simulink model "Sm_Ideal"  (R2025b)
settings: Solver=FixedStepDiscrete  StartTime=0.0  StopTime=0.1  FixedStep=Par_Sw_cdTs  RelTol=1e-3
undefined symbols (not defined in the file or in its folder): Par_Mtr_cfFlux, Par_Mtr_cfLd, Par_Mtr_cfLq, Par_Mtr_cfRs, Par_Mtr_cuNp, Par_Sw_cdTs
libraries: Lib_PMSMCtrl x3, eeTransforms x2
settings Model: DataDictionary=Sm_Ideal.sldd  SimulationMode=accelerator  Creator=62555  LastModifiedBy=62555
settings OptimizationCC: DefaultParameterBehavior=Inlined  UseDivisionForNetSlopeComputation=on  EnhancedBackFolding=on  PassReuseOutputArgsAs=Individual arguments  ZeroExternalMemoryAtStartup=off  ZeroInternalMemoryAtStartup=off  OptimizeBlockOrder=speed  DifferentSizesBufferReuse=on  OptimizationCustomize=off  EfficientTunableParamExpr=on
settings DebuggingCC: ParameterTunabilityLossMsg=error
settings SFSimCC: MATLABDynamicMemAlloc=off
settings RTWCC: SystemTargetFile=ert.tlc  GenCodeOnly=on  TemplateMakefile=ert_default_tmf  Toolchain=MinGW64 | gmake (64-bit Windows)  Description=Embedded Coder
settings CodeAppCC: ForceParamTrailComments=on  IgnoreCustomStorageClasses=off  OperatorAnnotations=on  SimulinkDataObjDesc=on  SFDataObjDesc=on  InsertBlockDesc=on
settings ERTTargetCC: ERTCustomFileTemplate=example_file_process.tlc  TargetLangStandard=C99 (ISO)  GenerateSampleERTMain=on

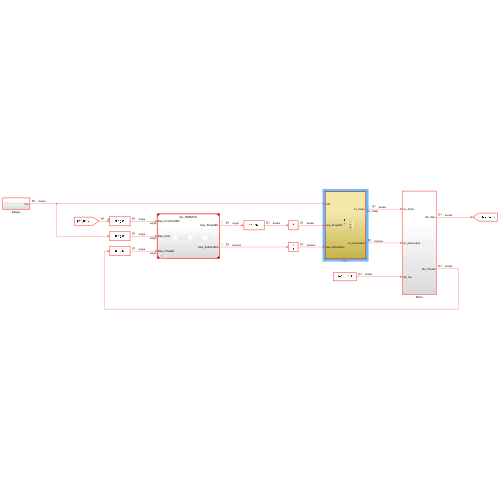
[thumbnail: Simulink's stored preview of the top-level diagram]
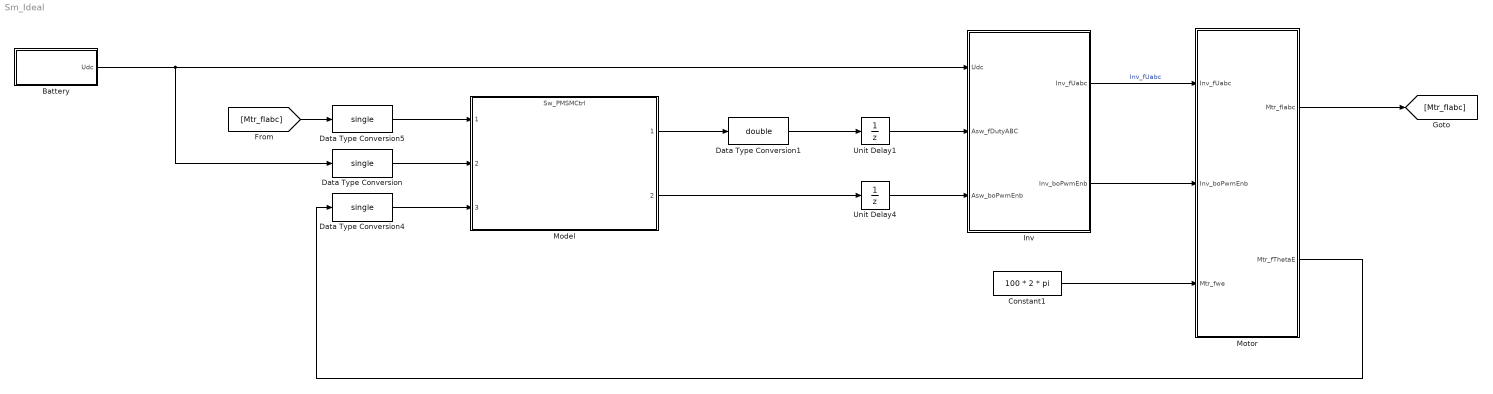
== system Sm_Ideal ==
  Battery : Subsystem
  Constant1 : Constant  Value=100 * 2 * pi  OutDataTypeStr=double  SampleTime=-1
  Data Type Conversion : DataTypeConversion  OutDataTypeStr=single  SaturateOnIntegerOverflow=off  RndMeth=Floor
  Data Type Conversion1 : DataTypeConversion  OutDataTypeStr=double  SaturateOnIntegerOverflow=off  RndMeth=Floor
  Data Type Conversion4 : DataTypeConversion  OutDataTypeStr=single  SaturateOnIntegerOverflow=off  RndMeth=Floor
  Data Type Conversion5 : DataTypeConversion  OutDataTypeStr=single  SaturateOnIntegerOverflow=off  RndMeth=Floor
  Inv : Subsystem
  Model : ModelReference  ModelNameDialog=Sw_PMSMCtrl.slx  ModelReferenceVersion=6.14
  Motor : Subsystem
  Unit Delay1 : UnitDelay  SampleTime=-1  HasFrameUpgradeWarning=on
  Unit Delay4 : UnitDelay  SampleTime=-1  HasFrameUpgradeWarning=on
  wires:
  Model/2 -> Unit Delay4/1
  Model/1 -> Data Type Conversion1/1
  Data Type Conversion/1 -> Model/2
  Data Type Conversion1/1 -> Unit Delay1/1
  Data Type Conversion4/1 -> Model/3
  Inv/2(Inv_boPwmEnb) -> Motor/2(Inv_boPwmEnb)
  Inv/1(Inv_fUabc) -> Motor/1(Inv_fUabc)  "Inv_fUabc"
  [Mtr_fIabc] -> Data Type Conversion5/1
  Data Type Conversion5/1 -> Model/1
  Motor/1(Mtr_fIabc) -> [Mtr_fIabc]
  Unit Delay1/1 -> Inv/2(Asw_fDutyABC)
  Unit Delay4/1 -> Inv/3(Asw_boPwmEnb)
  Battery/1(Udc) -> Inv/1(Udc), Data Type Conversion/1
  Constant1/1 -> Motor/3(Mtr_fwe)
  Motor/2(Mtr_fThetaE) -> Data Type Conversion4/1

== system Sm_Ideal/Battery ==
  Constant : Constant  Value=48  OutDataTypeStr=double  SampleTime=-1
  Udc : Outport
  wires:
  Constant/1 -> Udc/1

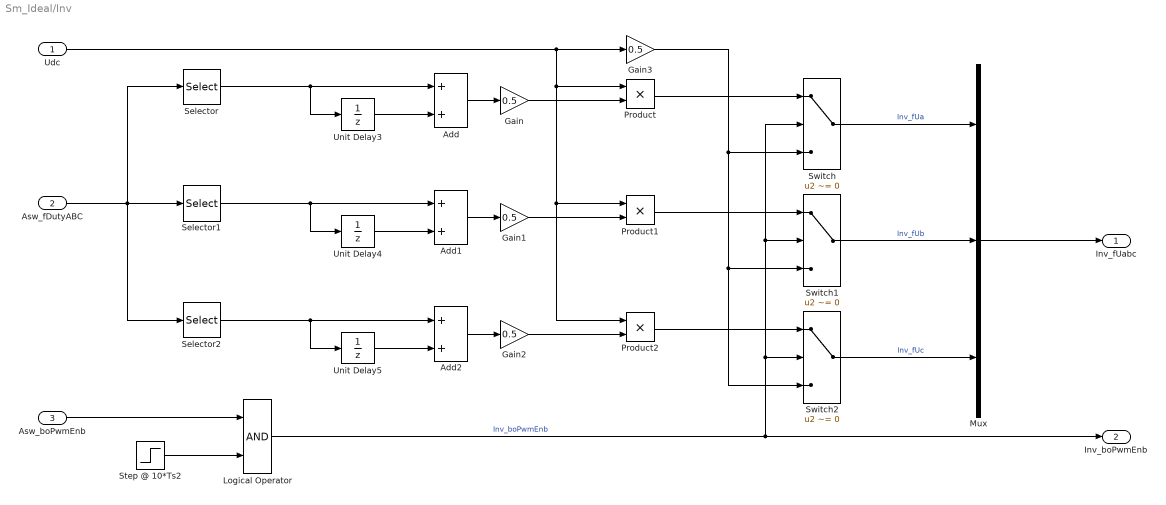
== system Sm_Ideal/Inv ==
  Udc : Inport
  Asw_fDutyABC : Inport  Port=2
  Asw_boPwmEnb : Inport  Port=3
  Add : Sum
  Add1 : Sum
  Add2 : Sum
  Gain{,1..3} (4 alike) : Gain  Gain=0.5
  Logical Operator : Logic  AllPortsSameDT=off  OutDataTypeStr=boolean
  Mux : Mux  Inputs=3
  Product : Product
  Product1 : Product
  Product2 : Product
  Selector : Selector  InputPortWidth=3  IndexOptions=Index vector (dialog)  Indices=[1]  OutputSizes=1
  Selector1 : Selector  InputPortWidth=3  IndexOptions=Index vector (dialog)  Indices=[2]  OutputSizes=1
  Selector2 : Selector  InputPortWidth=3  IndexOptions=Index vector (dialog)  Indices=[3]  OutputSizes=1
  Step @ 10*Ts2 : Step  Time=0.00050  SampleTime=Par_Sw_cdTs
  Switch : Switch  Criteria=u2 ~= 0  SaturateOnIntegerOverflow=off  InputSameDT=off
  Switch1 : Switch  Criteria=u2 ~= 0  SaturateOnIntegerOverflow=off  InputSameDT=off
  Switch2 : Switch  Criteria=u2 ~= 0  SaturateOnIntegerOverflow=off  InputSameDT=off
  Unit Delay3 : UnitDelay  SampleTime=-1  HasFrameUpgradeWarning=on
  Unit Delay4 : UnitDelay  SampleTime=-1  HasFrameUpgradeWarning=on
  Unit Delay5 : UnitDelay  SampleTime=-1  HasFrameUpgradeWarning=on
  Inv_fUabc : Outport
  Inv_boPwmEnb : Outport  Port=2
  wires:
  Udc/1 -> Gain3/1, Product2/1, Product1/1, Product/1
  Add/1 -> Gain/1
  Gain/1 -> Product/2
  Unit Delay3/1 -> Add/2
  Add1/1 -> Gain1/1
  Unit Delay4/1 -> Add1/2
  Add2/1 -> Gain2/1
  Unit Delay5/1 -> Add2/2
  Asw_fDutyABC/1 -> Selector/1, Selector2/1, Selector1/1
  Gain1/1 -> Product1/2
  Gain2/1 -> Product2/2
  Product/1 -> Switch/1
  Product1/1 -> Switch1/1
  Product2/1 -> Switch2/1
  Asw_boPwmEnb/1 -> Logical Operator/1
  Step @ 10*Ts2/1 -> Logical Operator/2
  Logical Operator/1 -> Switch1/2, Switch/2, Switch2/2, Inv_boPwmEnb/1  "Inv_boPwmEnb"
  Gain3/1 -> Switch2/3, Switch1/3, Switch/3
  Switch/1 -> Mux/1  "Inv_fUa"
  Switch2/1 -> Mux/3  "Inv_fUc"
  Switch1/1 -> Mux/2  "Inv_fUb"
  Mux/1 -> Inv_fUabc/1
  Selector/1 -> Unit Delay3/1, Add/1
  Selector1/1 -> Unit Delay4/1, Add1/1
  Selector2/1 -> Unit Delay5/1, Add2/1

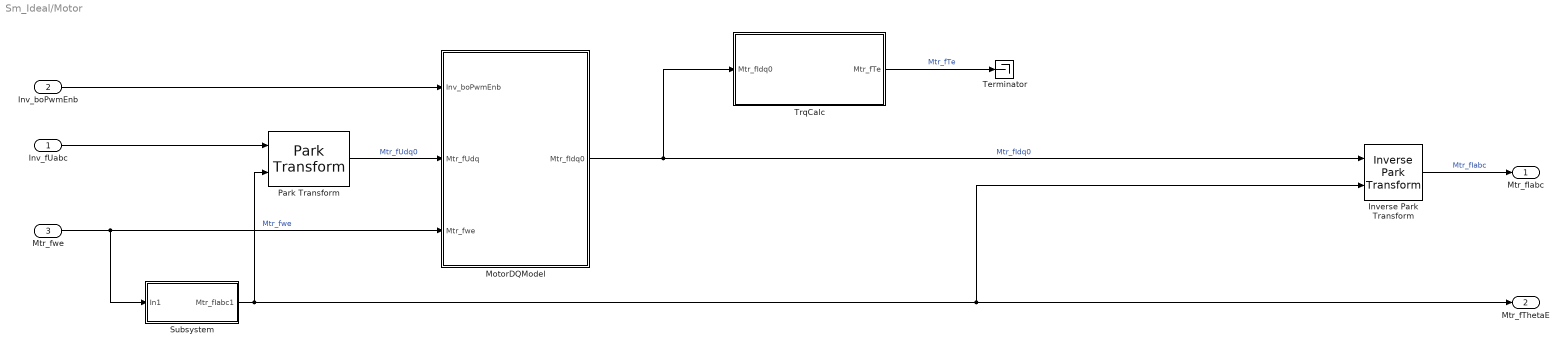
== system Sm_Ideal/Motor ==
  Inv_fUabc : Inport
  Inv_boPwmEnb : Inport  Port=2
  Mtr_fwe : Inport  Port=3
  Inverse Park Transform : eeTransforms/Inverse Park Transform  AxisAlignment=D-axis  PowerInvariant=off
      settings: LibrarySourceBlock=|
      | ee_sl_lib/Mathematical
      | Transforms/Inverse
      | Park Transform
  MotorDQModel : Subsystem  mask{Ld=Par_Mtr_cfLd, Lq=Par_Mtr_cfLq, Rs=Par_Mtr_cfRs, Psif=Par_Mtr_cfFlux}
      mask prompts: Ld "Ld (H)"; Lq "Lq (H)"; Rs "Rs (Ω)"; Psif "Psif (Wb)"
      mask Display:
      | disp('Motor Elec Model\n dq-Axis');
      | port_label('input',1, 'PwmEnb','interpreter', 'tex');
      | port_label('input',2, 'Udq0','interpreter', 'tex');
      | port_label('input',3, '\omega_e','interpreter', 'tex');
      | port_label('output',1, 'Idq0','interpreter', 'tex');
  Park Transform : eeTransforms/Park Transform  AxisAlignment=D-axis  PowerInvariant=off
      settings: LibrarySourceBlock=|
      | ee_sl_lib/Mathematical
      | Transforms/Park Transform
  Subsystem : Subsystem
  Terminator : Terminator
  TrqCalc : Subsystem
  Mtr_fIabc : Outport
  Mtr_fThetaE : Outport  Port=2
  wires:
  Mtr_fwe/1 -> Subsystem/1(In1), MotorDQModel/3(Mtr_fwe)  "Mtr_fwe"
  MotorDQModel/1(Mtr_fIdq0) -> TrqCalc/1(Mtr_fIdq0), Inverse Park Transform/1  "Mtr_fIdq0"
  Inv_boPwmEnb/1 -> MotorDQModel/1(Inv_boPwmEnb)
  Inv_fUabc/1 -> Park Transform/1
  Park Transform/1 -> MotorDQModel/2(Mtr_fUdq)  "Mtr_fUdq0"
  Inverse Park Transform/1 -> Mtr_fIabc/1  "Mtr_fIabc"
  TrqCalc/1(Mtr_fTe) -> Terminator/1  "Mtr_fTe"
  Subsystem/1(Mtr_fIabc1) -> Park Transform/2, Inverse Park Transform/2, Mtr_fThetaE/1

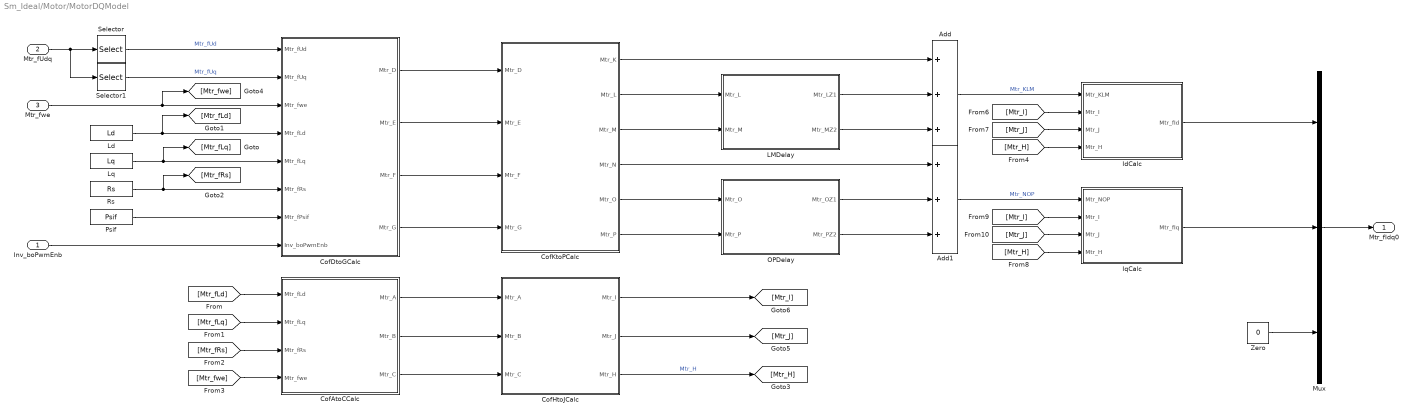
== system Sm_Ideal/Motor/MotorDQModel ==
  Inv_boPwmEnb : Inport
  Mtr_fUdq : Inport  Port=2
  Mtr_fwe : Inport  Port=3
  Add : Sum  Inputs=+++
  Add1 : Sum  Inputs=+++
  CofAtoCCalc : Subsystem
  CofDtoGCalc : Subsystem
  CofHtoJCalc : Subsystem
  CofKtoPCalc : Subsystem
  IdCalc : Subsystem
  IqCalc : Subsystem
  LMDelay : Subsystem
  Ld : Constant  Value=Ld  OutDataTypeStr=double  SampleTime=-1
  Lq : Constant  Value=Lq  OutDataTypeStr=double  SampleTime=-1
  Mux : Mux  Inputs=3
  OPDelay : Subsystem
  Psif : Constant  Value=Psif  OutDataTypeStr=double  SampleTime=-1
  Rs : Constant  Value=Rs  OutDataTypeStr=double  SampleTime=-1
  Selector : Selector  InputPortWidth=3  IndexOptions=Index vector (dialog)  Indices=[1]  OutputSizes=1
  Selector1 : Selector  InputPortWidth=3  IndexOptions=Index vector (dialog)  Indices=[2]  OutputSizes=1
  Zero : Constant  Value=0  OutDataTypeStr=Inherit: Inherit via back propagation
  Mtr_fIdq0 : Outport
  wires:
  [Mtr_fLd] -> CofAtoCCalc/1(Mtr_fLd)
  [Mtr_fLq] -> CofAtoCCalc/2(Mtr_fLq)
  [Mtr_fRs] -> CofAtoCCalc/3(Mtr_fRs)
  [Mtr_fwe] -> CofAtoCCalc/4(Mtr_fwe)
  Mtr_fwe/1 -> [Mtr_fwe], CofDtoGCalc/3(Mtr_fwe)
  Ld/1 -> CofDtoGCalc/4(Mtr_fLd), [Mtr_fLd]
  Lq/1 -> CofDtoGCalc/5(Mtr_fLq), [Mtr_fLq]
  Rs/1 -> [Mtr_fRs], CofDtoGCalc/6(Mtr_fRs)
  Psif/1 -> CofDtoGCalc/7(Mtr_fPsif)
  CofAtoCCalc/2(Mtr_B) -> CofHtoJCalc/2(Mtr_B)
  CofAtoCCalc/1(Mtr_A) -> CofHtoJCalc/1(Mtr_A)
  CofAtoCCalc/3(Mtr_C) -> CofHtoJCalc/3(Mtr_C)
  CofDtoGCalc/3(Mtr_F) -> CofKtoPCalc/3(Mtr_F)
  CofDtoGCalc/4(Mtr_G) -> CofKtoPCalc/4(Mtr_G)
  CofDtoGCalc/2(Mtr_E) -> CofKtoPCalc/2(Mtr_E)
  CofDtoGCalc/1(Mtr_D) -> CofKtoPCalc/1(Mtr_D)
  CofHtoJCalc/1(Mtr_I) -> [Mtr_I]
  CofHtoJCalc/2(Mtr_J) -> [Mtr_J]
  CofKtoPCalc/5(Mtr_O) -> OPDelay/1(Mtr_O)
  CofKtoPCalc/6(Mtr_P) -> OPDelay/2(Mtr_P)
  CofKtoPCalc/2(Mtr_L) -> LMDelay/1(Mtr_L)
  CofKtoPCalc/3(Mtr_M) -> LMDelay/2(Mtr_M)
  CofHtoJCalc/3(Mtr_H) -> [Mtr_H]  "Mtr_H"
  CofKtoPCalc/1(Mtr_K) -> Add/1
  CofKtoPCalc/4(Mtr_N) -> Add1/1
  LMDelay/1(Mtr_LZ1) -> Add/2
  LMDelay/2(Mtr_MZ2) -> Add/3
  OPDelay/1(Mtr_OZ1) -> Add1/2
  OPDelay/2(Mtr_PZ2) -> Add1/3
  Add/1 -> IdCalc/1(Mtr_KLM)  "Mtr_KLM"
  IdCalc/1(Mtr_fId) -> Mux/1
  [Mtr_H] -> IdCalc/4(Mtr_H)
  [Mtr_I] -> IdCalc/2(Mtr_I)
  [Mtr_J] -> IdCalc/3(Mtr_J)
  [Mtr_I] -> IqCalc/2(Mtr_I)
  [Mtr_J] -> IqCalc/3(Mtr_J)
  [Mtr_H] -> IqCalc/4(Mtr_H)
  Add1/1 -> IqCalc/1(Mtr_NOP)  "Mtr_NOP"
  IqCalc/1(Mtr_fIq) -> Mux/2
  Inv_boPwmEnb/1 -> CofDtoGCalc/8(Inv_boPwmEnb)
  Selector/1 -> CofDtoGCalc/1(Mtr_fUd)  "Mtr_fUd"
  Mtr_fUdq/1 -> Selector/1, Selector1/1
  Selector1/1 -> CofDtoGCalc/2(Mtr_fUq)  "Mtr_fUq"
  Mux/1 -> Mtr_fIdq0/1
  Zero/1 -> Mux/3

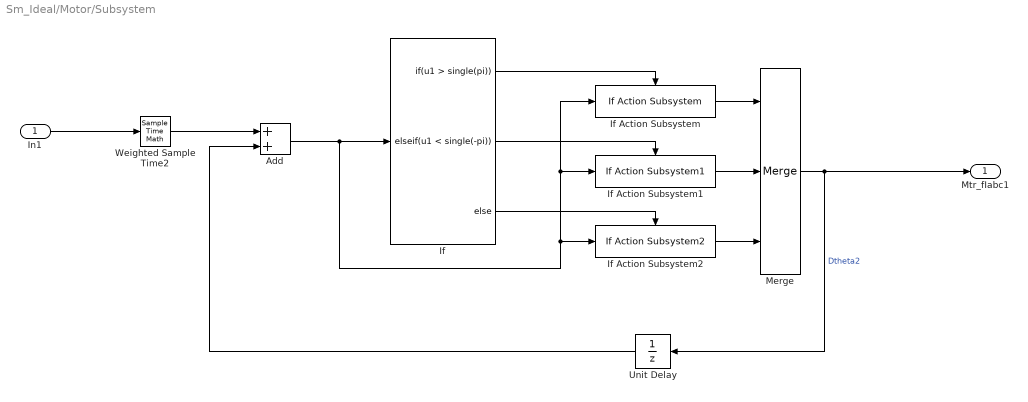
== system Sm_Ideal/Motor/Subsystem ==
  In1 : Inport
  Add : Sum
  If : If  IfExpression=u1 > single(pi)  ElseIfExpressions=u1 < single(-pi)
  If Action Subsystem : Lib_PMSMCtrl/PostoSpd/If Action Subsystem  SystemSampleTime=-1  VariantActivationTime=update diagram  EmptyChoice=off  PassThrough=off  PassThroughVariantControl=(default)  EmptyChoiceVariantControl=(default)  AllowFlexibleInterface=on  Latency=0  AutoFrameSizeCalculation=off
      settings: SourceProductName=Lib_PMSMCtrl
  If Action Subsystem1 : Lib_PMSMCtrl/PostoSpd/If Action Subsystem1  SystemSampleTime=-1  VariantActivationTime=update diagram  EmptyChoice=off  PassThrough=off  PassThroughVariantControl=(default)  EmptyChoiceVariantControl=(default)  AllowFlexibleInterface=on  Latency=0  AutoFrameSizeCalculation=off
      settings: SourceProductName=Lib_PMSMCtrl
  If Action Subsystem2 : Lib_PMSMCtrl/PostoSpd/If Action Subsystem2  SystemSampleTime=-1  VariantActivationTime=update diagram  EmptyChoice=off  PassThrough=off  PassThroughVariantControl=(default)  EmptyChoiceVariantControl=(default)  AllowFlexibleInterface=on  Latency=0  AutoFrameSizeCalculation=off
      settings: SourceProductName=Lib_PMSMCtrl
  Merge : Merge  Inputs=3
  Unit Delay : UnitDelay  SampleTime=-1  HasFrameUpgradeWarning=on
  Weighted Sample Time2 : SampleTimeMath  TsampMathOp=*
  Mtr_fIabc1 : Outport
  wires:
  If/3 -> If Action Subsystem2/Action
  If Action Subsystem/1 -> Merge/1
  If/2 -> If Action Subsystem1/Action
  Merge/1 -> Mtr_fIabc1/1, Unit Delay/1  "Dtheta2"
  If Action Subsystem2/1 -> Merge/3
  Weighted Sample Time2/1 -> Add/1
  Add/1 -> If Action Subsystem/1, If Action Subsystem1/1, If Action Subsystem2/1, If/1
  If/1 -> If Action Subsystem/Action
  If Action Subsystem1/1 -> Merge/2
  Unit Delay/1 -> Add/2
  In1/1 -> Weighted Sample Time2/1

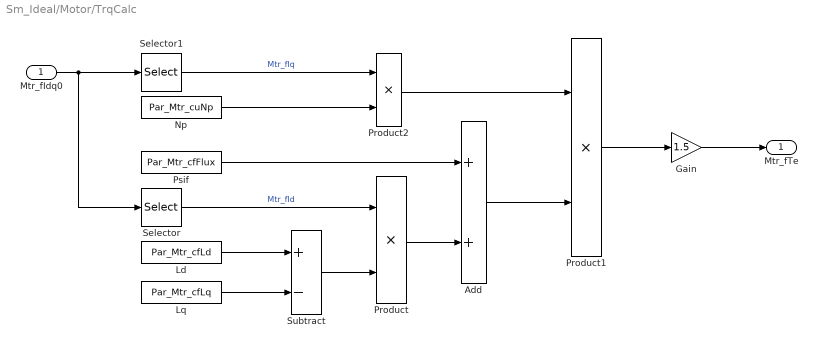
== system Sm_Ideal/Motor/TrqCalc ==
  Mtr_fIdq0 : Inport
  Add : Sum
  Gain : Gain  Gain=1.5
  Ld : Constant  Value=Par_Mtr_cfLd  OutDataTypeStr=double  SampleTime=-1
  Lq : Constant  Value=Par_Mtr_cfLq  OutDataTypeStr=double  SampleTime=-1
  Np : Constant  Value=Par_Mtr_cuNp  OutDataTypeStr=double  SampleTime=-1
  Product : Product
  Product1 : Product
  Product2 : Product
  Psif : Constant  Value=Par_Mtr_cfFlux  OutDataTypeStr=double  SampleTime=-1
  Selector : Selector  InputPortWidth=3  IndexOptions=Index vector (dialog)  Indices=[1]  OutputSizes=1
  Selector1 : Selector  InputPortWidth=3  IndexOptions=Index vector (dialog)  Indices=[2]  OutputSizes=1
  Subtract : Sum  Inputs=+-
  Mtr_fTe : Outport
  wires:
  Selector/1 -> Product/1  "Mtr_fId"
  Selector1/1 -> Product2/1  "Mtr_fIq"
  Mtr_fIdq0/1 -> Selector/1, Selector1/1
  Ld/1 -> Subtract/1
  Lq/1 -> Subtract/2
  Subtract/1 -> Product/2
  Product/1 -> Add/2
  Psif/1 -> Add/1
  Add/1 -> Product1/2
  Product1/1 -> Gain/1
  Gain/1 -> Mtr_fTe/1
  Product2/1 -> Product1/1
  Np/1 -> Product2/2

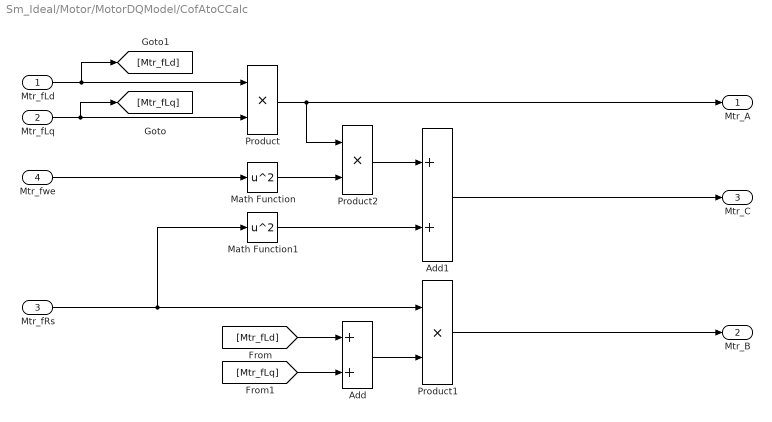
== system Sm_Ideal/Motor/MotorDQModel/CofAtoCCalc ==
  Mtr_fLd : Inport
  Mtr_fLq : Inport  Port=2
  Mtr_fRs : Inport  Port=3
  Mtr_fwe : Inport  Port=4
  Add : Sum
  Add1 : Sum
  Math Function : Math  Operator=square
  Math Function1 : Math  Operator=square
  Product : Product
  Product1 : Product
  Product2 : Product
  Mtr_A : Outport
  Mtr_B : Outport  Port=2
  Mtr_C : Outport  Port=3
  wires:
  Mtr_fLq/1 -> [Mtr_fLq], Product/2
  Mtr_fRs/1 -> Product1/1, Math Function1/1
  Product1/1 -> Mtr_B/1
  Mtr_fLd/1 -> [Mtr_fLd], Product/1
  Add1/1 -> Mtr_C/1
  Add/1 -> Product1/2
  [Mtr_fLd] -> Add/1
  [Mtr_fLq] -> Add/2
  Product2/1 -> Add1/1
  Mtr_fwe/1 -> Math Function/1
  Math Function/1 -> Product2/2
  Math Function1/1 -> Add1/2
  Product/1 -> Mtr_A/1, Product2/1

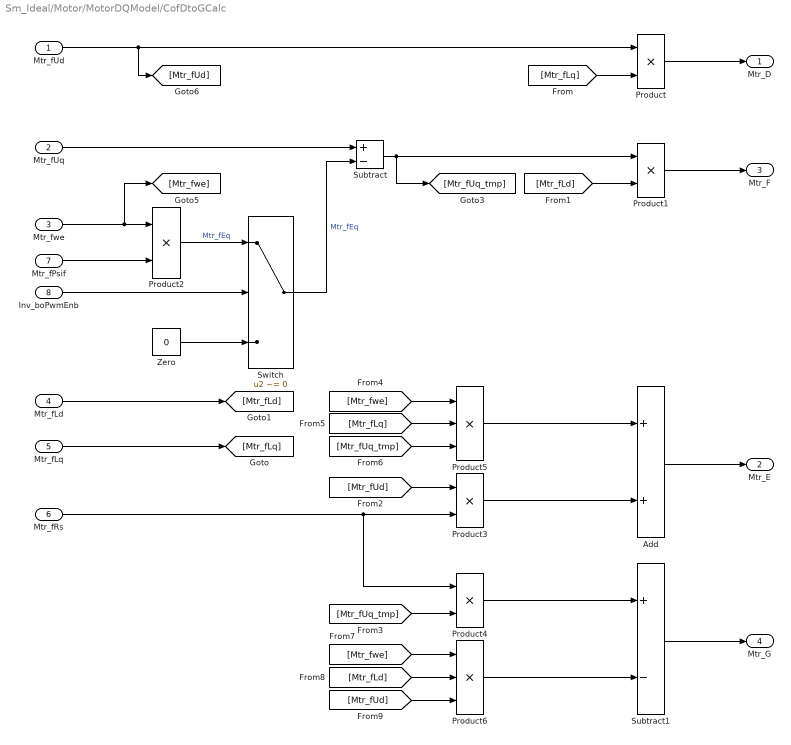
== system Sm_Ideal/Motor/MotorDQModel/CofDtoGCalc ==
  Mtr_fUd : Inport
  Mtr_fUq : Inport  Port=2
  Mtr_fwe : Inport  Port=3
  Mtr_fLd : Inport  Port=4
  Mtr_fLq : Inport  Port=5
  Mtr_fRs : Inport  Port=6
  Mtr_fPsif : Inport  Port=7
  Inv_boPwmEnb : Inport  Port=8
  Add : Sum
  Product{,1..4} (5 alike) : Product
  Product5 : Product  Inputs=3
  Product6 : Product  Inputs=3
  Subtract : Sum  Inputs=+-
  Subtract1 : Sum  Inputs=+-
  Switch : Switch  Criteria=u2 ~= 0  SaturateOnIntegerOverflow=off  InputSameDT=off
  Zero : Constant  Value=0  OutDataTypeStr=Inherit: Inherit via back propagation  SampleTime=-1
  Mtr_D : Outport
  Mtr_E : Outport  Port=2
  Mtr_F : Outport  Port=3
  Mtr_G : Outport  Port=4
  wires:
  Mtr_fLq/1 -> [Mtr_fLq]
  Mtr_fUd/1 -> Product/1, [Mtr_fUd]
  [Mtr_fLq] -> Product/2
  Product/1 -> Mtr_D/1
  Product1/1 -> Mtr_F/1
  Mtr_fLd/1 -> [Mtr_fLd]
  [Mtr_fLd] -> Product1/2
  Mtr_fwe/1 -> [Mtr_fwe], Product2/1
  Mtr_fPsif/1 -> Product2/2
  Switch/1 -> Subtract/2  "Mtr_fEq"
  Mtr_fUq/1 -> Subtract/1
  Subtract/1 -> Product1/1, [Mtr_fUq_tmp]
  [Mtr_fUd] -> Product3/1
  Mtr_fRs/1 -> Product4/1, Product3/2
  [Mtr_fUq_tmp] -> Product4/2
  Product3/1 -> Add/2
  Add/1 -> Mtr_E/1
  [Mtr_fwe] -> Product5/1
  Product5/1 -> Add/1
  [Mtr_fLq] -> Product5/2
  [Mtr_fUq_tmp] -> Product5/3
  Product4/1 -> Subtract1/1
  Subtract1/1 -> Mtr_G/1
  Product6/1 -> Subtract1/2
  [Mtr_fwe] -> Product6/1
  [Mtr_fLd] -> Product6/2
  [Mtr_fUd] -> Product6/3
  Product2/1 -> Switch/1  "Mtr_fEq"
  Inv_boPwmEnb/1 -> Switch/2
  Zero/1 -> Switch/3

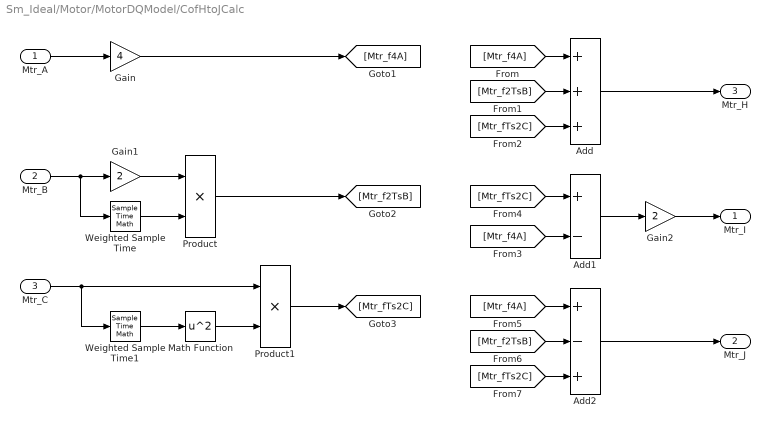
== system Sm_Ideal/Motor/MotorDQModel/CofHtoJCalc ==
  Mtr_A : Inport
  Mtr_B : Inport  Port=2
  Mtr_C : Inport  Port=3
  Add : Sum  Inputs=+++
  Add1 : Sum  Inputs=+-
  Add2 : Sum  Inputs=+-+
  Gain : Gain  Gain=4
  Gain1 : Gain  Gain=2
  Gain2 : Gain  Gain=2
  Math Function : Math  Operator=square
  Product : Product
  Product1 : Product
  Weighted Sample Time : SampleTimeMath  TsampMathOp=Ts Only
  Weighted Sample Time1 : SampleTimeMath  TsampMathOp=Ts Only
  Mtr_I : Outport
  Mtr_J : Outport  Port=2
  Mtr_H : Outport  Port=3
  wires:
  Mtr_B/1 -> Gain1/1, Weighted Sample Time/1
  Mtr_A/1 -> Gain/1
  Gain1/1 -> Product/1
  Weighted Sample Time/1 -> Product/2
  Mtr_C/1 -> Product1/1, Weighted Sample Time1/1
  Weighted Sample Time1/1 -> Math Function/1
  Math Function/1 -> Product1/2
  Add/1 -> Mtr_H/1
  Add1/1 -> Gain2/1
  Gain/1 -> [Mtr_f4A]
  Product/1 -> [Mtr_f2TsB]
  Product1/1 -> [Mtr_fTs2C]
  [Mtr_f4A] -> Add/1
  [Mtr_f2TsB] -> Add/2
  [Mtr_fTs2C] -> Add/3
  [Mtr_fTs2C] -> Add1/1
  [Mtr_f4A] -> Add1/2
  Add2/1 -> Mtr_J/1
  [Mtr_f4A] -> Add2/1
  [Mtr_f2TsB] -> Add2/2
  [Mtr_fTs2C] -> Add2/3
  Gain2/1 -> Mtr_I/1

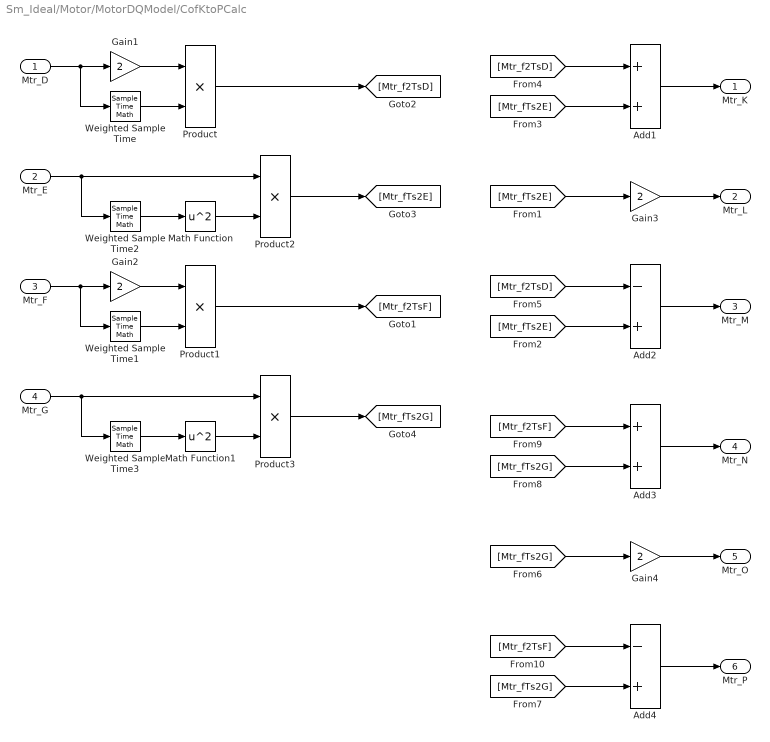
== system Sm_Ideal/Motor/MotorDQModel/CofKtoPCalc ==
  Mtr_D : Inport
  Mtr_E : Inport  Port=2
  Mtr_F : Inport  Port=3
  Mtr_G : Inport  Port=4
  Add1 : Sum
  Add2 : Sum  Inputs=-+
  Add3 : Sum
  Add4 : Sum  Inputs=-+
  Gain{1..4} (4 alike) : Gain  Gain=2
  Math Function : Math  Operator=square
  Math Function1 : Math  Operator=square
  Product{,1..3} (4 alike) : Product
  Weighted Sample Time{,1..3} (4 alike) : SampleTimeMath  TsampMathOp=Ts Only
  Mtr_K : Outport
  Mtr_L : Outport  Port=2
  Mtr_M : Outport  Port=3
  Mtr_N : Outport  Port=4
  Mtr_O : Outport  Port=5
  Mtr_P : Outport  Port=6
  wires:
  Mtr_D/1 -> Gain1/1, Weighted Sample Time/1
  Weighted Sample Time/1 -> Product/2
  Product/1 -> [Mtr_f2TsD]
  Gain1/1 -> Product/1
  Gain2/1 -> Product1/1
  Weighted Sample Time1/1 -> Product1/2
  Mtr_F/1 -> Gain2/1, Weighted Sample Time1/1
  Product1/1 -> [Mtr_f2TsF]
  Weighted Sample Time2/1 -> Math Function/1
  Mtr_E/1 -> Product2/1, Weighted Sample Time2/1
  Product2/1 -> [Mtr_fTs2E]
  Math Function/1 -> Product2/2
  Mtr_G/1 -> Product3/1, Weighted Sample Time3/1
  Weighted Sample Time3/1 -> Math Function1/1
  Product3/1 -> [Mtr_fTs2G]
  Math Function1/1 -> Product3/2
  Add1/1 -> Mtr_K/1
  [Mtr_fTs2E] -> Gain3/1
  Gain3/1 -> Mtr_L/1
  [Mtr_f2TsD] -> Add1/1
  [Mtr_fTs2E] -> Add1/2
  [Mtr_fTs2E] -> Add2/2
  [Mtr_f2TsD] -> Add2/1
  Add2/1 -> Mtr_M/1
  [Mtr_f2TsF] -> Add4/1
  [Mtr_fTs2G] -> Add4/2
  [Mtr_f2TsF] -> Add3/1
  Add3/1 -> Mtr_N/1
  [Mtr_fTs2G] -> Gain4/1
  [Mtr_fTs2G] -> Add3/2
  Add4/1 -> Mtr_P/1
  Gain4/1 -> Mtr_O/1

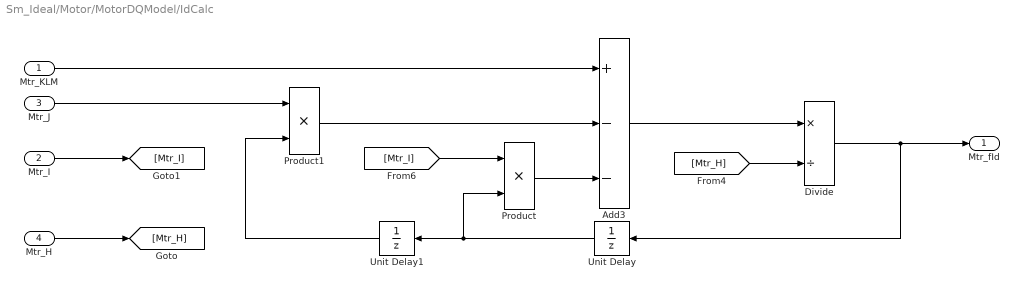
== system Sm_Ideal/Motor/MotorDQModel/IdCalc ==
  Mtr_KLM : Inport
  Mtr_I : Inport  Port=2
  Mtr_J : Inport  Port=3
  Mtr_H : Inport  Port=4
  Add3 : Sum  Inputs=+--
  Divide : Product  Inputs=*/
  Product : Product
  Product1 : Product
  Unit Delay : UnitDelay  SampleTime=-1  HasFrameUpgradeWarning=on
  Unit Delay1 : UnitDelay  SampleTime=-1  HasFrameUpgradeWarning=on
  Mtr_fId : Outport
  wires:
  Product/1 -> Add3/3
  Mtr_KLM/1 -> Add3/1
  Unit Delay/1 -> Product/2, Unit Delay1/1
  Divide/1 -> Mtr_fId/1, Unit Delay/1
  Add3/1 -> Divide/1
  [Mtr_H] -> Divide/2
  Product1/1 -> Add3/2
  [Mtr_I] -> Product/1
  Unit Delay1/1 -> Product1/2
  Mtr_H/1 -> [Mtr_H]
  Mtr_I/1 -> [Mtr_I]
  Mtr_J/1 -> Product1/1

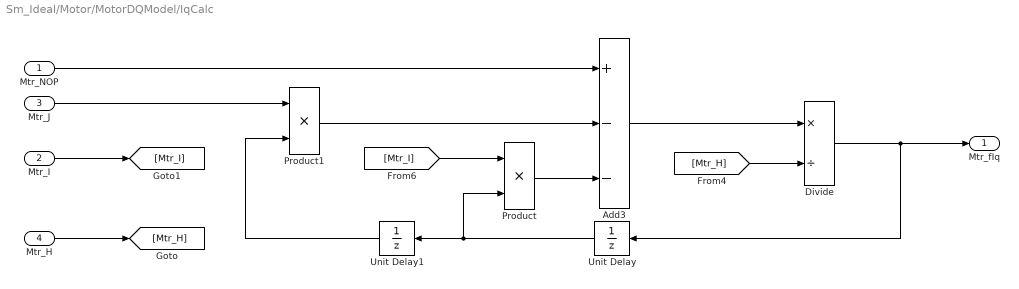
== system Sm_Ideal/Motor/MotorDQModel/IqCalc ==
  Mtr_NOP : Inport
  Mtr_I : Inport  Port=2
  Mtr_J : Inport  Port=3
  Mtr_H : Inport  Port=4
  Add3 : Sum  Inputs=+--
  Divide : Product  Inputs=*/
  Product : Product
  Product1 : Product
  Unit Delay : UnitDelay  SampleTime=-1  HasFrameUpgradeWarning=on
  Unit Delay1 : UnitDelay  SampleTime=-1  HasFrameUpgradeWarning=on
  Mtr_fIq : Outport
  wires:
  Product/1 -> Add3/3
  Mtr_NOP/1 -> Add3/1
  Unit Delay/1 -> Product/2, Unit Delay1/1
  Divide/1 -> Mtr_fIq/1, Unit Delay/1
  Add3/1 -> Divide/1
  [Mtr_H] -> Divide/2
  Product1/1 -> Add3/2
  [Mtr_I] -> Product/1
  Unit Delay1/1 -> Product1/2
  Mtr_H/1 -> [Mtr_H]
  Mtr_I/1 -> [Mtr_I]
  Mtr_J/1 -> Product1/1

== system Sm_Ideal/Motor/MotorDQModel/LMDelay ==
  Mtr_L : Inport
  Mtr_M : Inport  Port=2
  Unit Delay : UnitDelay  SampleTime=-1  HasFrameUpgradeWarning=on
  Unit Delay1 : UnitDelay  SampleTime=-1  HasFrameUpgradeWarning=on
  Unit Delay2 : UnitDelay  SampleTime=-1  HasFrameUpgradeWarning=on
  Mtr_LZ1 : Outport
  Mtr_MZ2 : Outport  Port=2
  wires:
  Mtr_L/1 -> Unit Delay/1
  Mtr_M/1 -> Unit Delay1/1
  Unit Delay/1 -> Mtr_LZ1/1
  Unit Delay1/1 -> Unit Delay2/1
  Unit Delay2/1 -> Mtr_MZ2/1

== system Sm_Ideal/Motor/MotorDQModel/OPDelay ==
  Mtr_O : Inport
  Mtr_P : Inport  Port=2
  Unit Delay : UnitDelay  SampleTime=-1  HasFrameUpgradeWarning=on
  Unit Delay1 : UnitDelay  SampleTime=-1  HasFrameUpgradeWarning=on
  Unit Delay2 : UnitDelay  SampleTime=-1  HasFrameUpgradeWarning=on
  Mtr_OZ1 : Outport
  Mtr_PZ2 : Outport  Port=2
  wires:
  Mtr_O/1 -> Unit Delay/1
  Mtr_P/1 -> Unit Delay1/1
  Unit Delay/1 -> Mtr_OZ1/1
  Unit Delay1/1 -> Unit Delay2/1
  Unit Delay2/1 -> Mtr_PZ2/1
